simulink model "pid_anti_windup_back_calculation"  (R2026b)
settings: Solver=ode4  StopTime=30  FixedStep=0.05
settings Model: Creator=ZAID  LastModifiedBy=ZAID

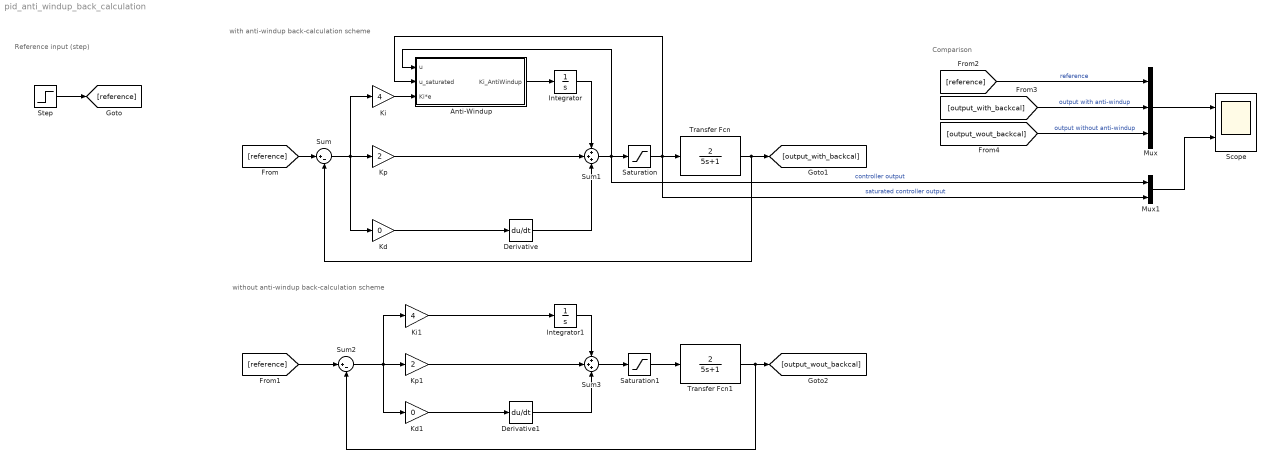
== system pid_anti_windup_back_calculation ==
  note: Comparison
  note: Reference input (step)
  note: with anti-windup back-calculation scheme
  note: without anti-windup back-calculation scheme
  Anti-Windup : Subsystem
  Derivative : Derivative
  Derivative1 : Derivative
  Integrator : Integrator
  Integrator1 : Integrator
  Kd : Gain  Gain=0
  Kd1 : Gain  Gain=0
  Ki : Gain  Gain=4
  Ki1 : Gain  Gain=4
  Kp : Gain  Gain=2
  Kp1 : Gain  Gain=2
  Mux : Mux  Inputs=3
  Mux1 : Mux  Inputs=2
  Saturation : Saturate  UpperLimit=10  LowerLimit=-10
      settings: AttributesFormatString=|
      | u_max = %<UpperLimit>
      | u_min = %<LowerLimit>
  Saturation1 : Saturate  UpperLimit=10  LowerLimit=-10
      settings: AttributesFormatString=|
      | u_max = %<UpperLimit>
      | u_min = %<LowerLimit>
  Scope : Scope  NumInputPorts=2
      settings: ActiveDisplayYMinimum=-5.7211733189854082  ActiveDisplayYMaximum=51.49055987086868
  Step : Step  FinalValue=15  SampleTime=0
  Sum : Sum  Inputs=|+-
  Sum1 : Sum  Inputs=+++
  Sum2 : Sum  Inputs=|+-
  Sum3 : Sum  Inputs=+++
  Transfer Fcn : TransferFcn  Numerator=2  Denominator=[5 1]
  Transfer Fcn1 : TransferFcn  Numerator=2  Denominator=[5 1]
  wires:
  Sum/1 -> Ki/1, Kd/1, Kp/1
  Kd/1 -> Derivative/1
  Kp/1 -> Sum1/2
  Integrator/1 -> Sum1/1
  Derivative/1 -> Sum1/3
  Sum1/1 -> Anti-Windup/1(u), Mux1/1, Saturation/1  "controller output"
  Transfer Fcn/1 -> [output_with_backcal], Sum/2
  Saturation/1 -> Anti-Windup/2(u_saturated), Mux1/2, Transfer Fcn/1  "saturated controller output"
  Anti-Windup/1(Ki_AntiWindup) -> Integrator/1
  Ki/1 -> Anti-Windup/3(Ki*e)
  Ki1/1 -> Integrator1/1
  Saturation1/1 -> Transfer Fcn1/1
  Transfer Fcn1/1 -> Sum2/2, [output_wout_backcal]
  Sum3/1 -> Saturation1/1
  Derivative1/1 -> Sum3/3
  Integrator1/1 -> Sum3/1
  Kp1/1 -> Sum3/2
  Kd1/1 -> Derivative1/1
  Sum2/1 -> Kp1/1, Kd1/1, Ki1/1
  Step/1 -> [reference]
  [reference] -> Sum/1
  [reference] -> Sum2/1
  [reference] -> Mux/1  "reference"
  [output_with_backcal] -> Mux/2  "output with anti-windup"
  [output_wout_backcal] -> Mux/3  "output without anti-windup"
  Mux/1 -> Scope/1
  Mux1/1 -> Scope/2

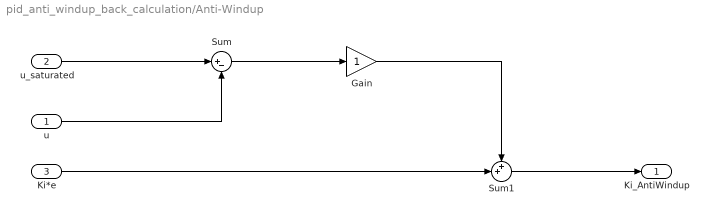
== system pid_anti_windup_back_calculation/Anti-Windup ==
  u : Inport
  u_saturated : Inport  Port=2
  Ki*e : Inport  Port=3
  Gain : Gain
  Sum : Sum  Inputs=|+-
  Sum1 : Sum  Inputs=++|
  Ki_AntiWindup : Outport
  wires:
  u/1 -> Sum/2
  Ki*e/1 -> Sum1/2
  Sum1/1 -> Ki_AntiWindup/1
  u_saturated/1 -> Sum/1
  Sum/1 -> Gain/1
  Gain/1 -> Sum1/1
